simulink model "Hexapod_PD"  (R2026a)
settings: Solver=daessc  StopTime=ref.t(end)  FixedStep=2e-5
InitFcn:
  | startup
model workspace: external: MATLAB File Hexapod_DataFile.m (data not in the file)
undefined symbols (not defined in the file or in its folder): ref, robot, smiData, vc, X, Y, Z
libraries: sm_lib x805, nesl_utility x43
(part 11 of 15)

== system Hexapod_PD/Base/Base_Side_a_2_RIGID/x90576A137_Medium_Strength_Steel_Nylon_Insert_Locknut_2_RIGID ==
  ReferenceFrame : sm_lib/Frames and Transforms/Reference Frame
  Solid : sm_lib/Body Elements/File Solid  ExtGeomFileName=90576A137_Medium-Strength Steel Nylon-Insert Locknut_90576A137_sldprt.STEP  UnitType=FromFile  ExtGeomFileUnits=m  StepReaderType=HEX  ExportConvexHullGeometry=off  InertiaType=Custom  BasedOnType=DensityFromFile  Density=1000  DensityUnits=kg/m^3  Mass=smiData.Solid(5).mass  MassUnits=kg  CenterOfMass=smiData.Solid(5).CoM  CenterOfMassUnits=mm  MomentsOfInertia=smiData.Solid(5).MoI  MomentsOfInertiaUnits=kg*mm^2  ProductsOfInertia=smiData.Solid(5).PoI  ProductsOfInertiaUnits=kg*mm^2  GraphicType=FromGeometry  MarkerShape=Sphere  MarkerSize=10  GraphicVisPropType=SimpleVisualProperties  GraphicDiffuseColor=smiData.Solid(5).color  GraphicOpacity=smiData.Solid(5).opacity  GraphicSpecularColor=[0.5 0.5 0.5 1.0]  GraphicAmbientColor=[0.15 0.15 0.15 1.0]  GraphicEmissiveColor=[0.0 0.0 0.0 1.0]  GraphicShininess=75  DoExposeReferenceFrame=on  SerializedFrames=<Frames/>
  F : PMIOPort  Side=Left
  connections:
  Solid/RConn1 -- ReferenceFrame/RConn1 -- F/RConn1

== system Hexapod_PD/Base/Base_Side_a_2_RIGID/x90576A137_Medium_Strength_Steel_Nylon_Insert_Locknut_3_RIGID ==
  ReferenceFrame : sm_lib/Frames and Transforms/Reference Frame
  Solid : sm_lib/Body Elements/File Solid  ExtGeomFileName=90576A137_Medium-Strength Steel Nylon-Insert Locknut_90576A137_sldprt.STEP  UnitType=FromFile  ExtGeomFileUnits=m  StepReaderType=HEX  ExportConvexHullGeometry=off  InertiaType=Custom  BasedOnType=DensityFromFile  Density=1000  DensityUnits=kg/m^3  Mass=smiData.Solid(5).mass  MassUnits=kg  CenterOfMass=smiData.Solid(5).CoM  CenterOfMassUnits=mm  MomentsOfInertia=smiData.Solid(5).MoI  MomentsOfInertiaUnits=kg*mm^2  ProductsOfInertia=smiData.Solid(5).PoI  ProductsOfInertiaUnits=kg*mm^2  GraphicType=FromGeometry  MarkerShape=Sphere  MarkerSize=10  GraphicVisPropType=SimpleVisualProperties  GraphicDiffuseColor=smiData.Solid(5).color  GraphicOpacity=smiData.Solid(5).opacity  GraphicSpecularColor=[0.5 0.5 0.5 1.0]  GraphicAmbientColor=[0.15 0.15 0.15 1.0]  GraphicEmissiveColor=[0.0 0.0 0.0 1.0]  GraphicShininess=75  DoExposeReferenceFrame=on  SerializedFrames=<Frames/>
  F : PMIOPort  Side=Left
  connections:
  Solid/RConn1 -- ReferenceFrame/RConn1 -- F/RConn1

== system Hexapod_PD/Base/Base_Side_a_2_RIGID/x90576A137_Medium_Strength_Steel_Nylon_Insert_Locknut_4_RIGID ==
  ReferenceFrame : sm_lib/Frames and Transforms/Reference Frame
  Solid : sm_lib/Body Elements/File Solid  ExtGeomFileName=90576A137_Medium-Strength Steel Nylon-Insert Locknut_90576A137_sldprt.STEP  UnitType=FromFile  ExtGeomFileUnits=m  StepReaderType=HEX  ExportConvexHullGeometry=off  InertiaType=Custom  BasedOnType=DensityFromFile  Density=1000  DensityUnits=kg/m^3  Mass=smiData.Solid(5).mass  MassUnits=kg  CenterOfMass=smiData.Solid(5).CoM  CenterOfMassUnits=mm  MomentsOfInertia=smiData.Solid(5).MoI  MomentsOfInertiaUnits=kg*mm^2  ProductsOfInertia=smiData.Solid(5).PoI  ProductsOfInertiaUnits=kg*mm^2  GraphicType=FromGeometry  MarkerShape=Sphere  MarkerSize=10  GraphicVisPropType=SimpleVisualProperties  GraphicDiffuseColor=smiData.Solid(5).color  GraphicOpacity=smiData.Solid(5).opacity  GraphicSpecularColor=[0.5 0.5 0.5 1.0]  GraphicAmbientColor=[0.15 0.15 0.15 1.0]  GraphicEmissiveColor=[0.0 0.0 0.0 1.0]  GraphicShininess=75  DoExposeReferenceFrame=on  SerializedFrames=<Frames/>
  F : PMIOPort  Side=Left
  connections:
  Solid/RConn1 -- ReferenceFrame/RConn1 -- F/RConn1

== system Hexapod_PD/Base/Base_Side_a_2_RIGID/x91259A710_Alloy_Steel_Shoulder_Screw_1_RIGID ==
  ReferenceFrame : sm_lib/Frames and Transforms/Reference Frame
  Solid : sm_lib/Body Elements/File Solid  ExtGeomFileName=91259A710_Alloy Steel Shoulder Screw_91259A710_sldprt.STEP  UnitType=FromFile  ExtGeomFileUnits=m  StepReaderType=HEX  ExportConvexHullGeometry=off  InertiaType=Custom  BasedOnType=DensityFromFile  Density=1000  DensityUnits=kg/m^3  Mass=smiData.Solid(4).mass  MassUnits=kg  CenterOfMass=smiData.Solid(4).CoM  CenterOfMassUnits=in  MomentsOfInertia=smiData.Solid(4).MoI  MomentsOfInertiaUnits=kg*in^2  ProductsOfInertia=smiData.Solid(4).PoI  ProductsOfInertiaUnits=kg*in^2  GraphicType=FromGeometry  MarkerShape=Sphere  MarkerSize=10  GraphicVisPropType=SimpleVisualProperties  GraphicDiffuseColor=smiData.Solid(4).color  GraphicOpacity=smiData.Solid(4).opacity  GraphicSpecularColor=[0.5 0.5 0.5 1.0]  GraphicAmbientColor=[0.15 0.15 0.15 1.0]  GraphicEmissiveColor=[0.0 0.0 0.0 1.0]  GraphicShininess=75  DoExposeReferenceFrame=on  SerializedFrames=<Frames/>
  F : PMIOPort  Side=Left
  connections:
  Solid/RConn1 -- ReferenceFrame/RConn1 -- F/RConn1

== system Hexapod_PD/Base/Base_Side_a_2_RIGID/x91259A710_Alloy_Steel_Shoulder_Screw_2_RIGID ==
  ReferenceFrame : sm_lib/Frames and Transforms/Reference Frame
  Solid : sm_lib/Body Elements/File Solid  ExtGeomFileName=91259A710_Alloy Steel Shoulder Screw_91259A710_sldprt.STEP  UnitType=FromFile  ExtGeomFileUnits=m  StepReaderType=HEX  ExportConvexHullGeometry=off  InertiaType=Custom  BasedOnType=DensityFromFile  Density=1000  DensityUnits=kg/m^3  Mass=smiData.Solid(4).mass  MassUnits=kg  CenterOfMass=smiData.Solid(4).CoM  CenterOfMassUnits=in  MomentsOfInertia=smiData.Solid(4).MoI  MomentsOfInertiaUnits=kg*in^2  ProductsOfInertia=smiData.Solid(4).PoI  ProductsOfInertiaUnits=kg*in^2  GraphicType=FromGeometry  MarkerShape=Sphere  MarkerSize=10  GraphicVisPropType=SimpleVisualProperties  GraphicDiffuseColor=smiData.Solid(4).color  GraphicOpacity=smiData.Solid(4).opacity  GraphicSpecularColor=[0.5 0.5 0.5 1.0]  GraphicAmbientColor=[0.15 0.15 0.15 1.0]  GraphicEmissiveColor=[0.0 0.0 0.0 1.0]  GraphicShininess=75  DoExposeReferenceFrame=on  SerializedFrames=<Frames/>
  F : PMIOPort  Side=Left
  connections:
  Solid/RConn1 -- ReferenceFrame/RConn1 -- F/RConn1

== system Hexapod_PD/Base/Base_Side_a_2_RIGID/x91259A710_Alloy_Steel_Shoulder_Screw_3_RIGID ==
  ReferenceFrame : sm_lib/Frames and Transforms/Reference Frame
  Solid : sm_lib/Body Elements/File Solid  ExtGeomFileName=91259A710_Alloy Steel Shoulder Screw_91259A710_sldprt.STEP  UnitType=FromFile  ExtGeomFileUnits=m  StepReaderType=HEX  ExportConvexHullGeometry=off  InertiaType=Custom  BasedOnType=DensityFromFile  Density=1000  DensityUnits=kg/m^3  Mass=smiData.Solid(4).mass  MassUnits=kg  CenterOfMass=smiData.Solid(4).CoM  CenterOfMassUnits=in  MomentsOfInertia=smiData.Solid(4).MoI  MomentsOfInertiaUnits=kg*in^2  ProductsOfInertia=smiData.Solid(4).PoI  ProductsOfInertiaUnits=kg*in^2  GraphicType=FromGeometry  MarkerShape=Sphere  MarkerSize=10  GraphicVisPropType=SimpleVisualProperties  GraphicDiffuseColor=smiData.Solid(4).color  GraphicOpacity=smiData.Solid(4).opacity  GraphicSpecularColor=[0.5 0.5 0.5 1.0]  GraphicAmbientColor=[0.15 0.15 0.15 1.0]  GraphicEmissiveColor=[0.0 0.0 0.0 1.0]  GraphicShininess=75  DoExposeReferenceFrame=on  SerializedFrames=<Frames/>
  F : PMIOPort  Side=Left
  connections:
  Solid/RConn1 -- ReferenceFrame/RConn1 -- F/RConn1

== system Hexapod_PD/Base/Base_Side_a_2_RIGID/x91259A710_Alloy_Steel_Shoulder_Screw_4_RIGID ==
  ReferenceFrame : sm_lib/Frames and Transforms/Reference Frame
  Solid : sm_lib/Body Elements/File Solid  ExtGeomFileName=91259A710_Alloy Steel Shoulder Screw_91259A710_sldprt.STEP  UnitType=FromFile  ExtGeomFileUnits=m  StepReaderType=HEX  ExportConvexHullGeometry=off  InertiaType=Custom  BasedOnType=DensityFromFile  Density=1000  DensityUnits=kg/m^3  Mass=smiData.Solid(4).mass  MassUnits=kg  CenterOfMass=smiData.Solid(4).CoM  CenterOfMassUnits=in  MomentsOfInertia=smiData.Solid(4).MoI  MomentsOfInertiaUnits=kg*in^2  ProductsOfInertia=smiData.Solid(4).PoI  ProductsOfInertiaUnits=kg*in^2  GraphicType=FromGeometry  MarkerShape=Sphere  MarkerSize=10  GraphicVisPropType=SimpleVisualProperties  GraphicDiffuseColor=smiData.Solid(4).color  GraphicOpacity=smiData.Solid(4).opacity  GraphicSpecularColor=[0.5 0.5 0.5 1.0]  GraphicAmbientColor=[0.15 0.15 0.15 1.0]  GraphicEmissiveColor=[0.0 0.0 0.0 1.0]  GraphicShininess=75  DoExposeReferenceFrame=on  SerializedFrames=<Frames/>
  F : PMIOPort  Side=Left
  connections:
  Solid/RConn1 -- ReferenceFrame/RConn1 -- F/RConn1

== system Hexapod_PD/Base/Base_Side_a_2_RIGID/x91259A710_Alloy_Steel_Shoulder_Screw_5_RIGID ==
  ReferenceFrame : sm_lib/Frames and Transforms/Reference Frame
  Solid : sm_lib/Body Elements/File Solid  ExtGeomFileName=91259A710_Alloy Steel Shoulder Screw_91259A710_sldprt.STEP  UnitType=FromFile  ExtGeomFileUnits=m  StepReaderType=HEX  ExportConvexHullGeometry=off  InertiaType=Custom  BasedOnType=DensityFromFile  Density=1000  DensityUnits=kg/m^3  Mass=smiData.Solid(4).mass  MassUnits=kg  CenterOfMass=smiData.Solid(4).CoM  CenterOfMassUnits=in  MomentsOfInertia=smiData.Solid(4).MoI  MomentsOfInertiaUnits=kg*in^2  ProductsOfInertia=smiData.Solid(4).PoI  ProductsOfInertiaUnits=kg*in^2  GraphicType=FromGeometry  MarkerShape=Sphere  MarkerSize=10  GraphicVisPropType=SimpleVisualProperties  GraphicDiffuseColor=smiData.Solid(4).color  GraphicOpacity=smiData.Solid(4).opacity  GraphicSpecularColor=[0.5 0.5 0.5 1.0]  GraphicAmbientColor=[0.15 0.15 0.15 1.0]  GraphicEmissiveColor=[0.0 0.0 0.0 1.0]  GraphicShininess=75  DoExposeReferenceFrame=on  SerializedFrames=<Frames/>
  F : PMIOPort  Side=Left
  connections:
  Solid/RConn1 -- ReferenceFrame/RConn1 -- F/RConn1

== system Hexapod_PD/Base/Base_Side_a_2_RIGID/x91259A710_Alloy_Steel_Shoulder_Screw_6_RIGID ==
  ReferenceFrame : sm_lib/Frames and Transforms/Reference Frame
  Solid : sm_lib/Body Elements/File Solid  ExtGeomFileName=91259A710_Alloy Steel Shoulder Screw_91259A710_sldprt.STEP  UnitType=FromFile  ExtGeomFileUnits=m  StepReaderType=HEX  ExportConvexHullGeometry=off  InertiaType=Custom  BasedOnType=DensityFromFile  Density=1000  DensityUnits=kg/m^3  Mass=smiData.Solid(4).mass  MassUnits=kg  CenterOfMass=smiData.Solid(4).CoM  CenterOfMassUnits=in  MomentsOfInertia=smiData.Solid(4).MoI  MomentsOfInertiaUnits=kg*in^2  ProductsOfInertia=smiData.Solid(4).PoI  ProductsOfInertiaUnits=kg*in^2  GraphicType=FromGeometry  MarkerShape=Sphere  MarkerSize=10  GraphicVisPropType=SimpleVisualProperties  GraphicDiffuseColor=smiData.Solid(4).color  GraphicOpacity=smiData.Solid(4).opacity  GraphicSpecularColor=[0.5 0.5 0.5 1.0]  GraphicAmbientColor=[0.15 0.15 0.15 1.0]  GraphicEmissiveColor=[0.0 0.0 0.0 1.0]  GraphicShininess=75  DoExposeReferenceFrame=on  SerializedFrames=<Frames/>
  F : PMIOPort  Side=Left
  connections:
  Solid/RConn1 -- ReferenceFrame/RConn1 -- F/RConn1

== system Hexapod_PD/Base/Base_Side_a_2_RIGID/x91259A710_Alloy_Steel_Shoulder_Screw_7_RIGID ==
  ReferenceFrame : sm_lib/Frames and Transforms/Reference Frame
  Solid : sm_lib/Body Elements/File Solid  ExtGeomFileName=91259A710_Alloy Steel Shoulder Screw_91259A710_sldprt.STEP  UnitType=FromFile  ExtGeomFileUnits=m  StepReaderType=HEX  ExportConvexHullGeometry=off  InertiaType=Custom  BasedOnType=DensityFromFile  Density=1000  DensityUnits=kg/m^3  Mass=smiData.Solid(4).mass  MassUnits=kg  CenterOfMass=smiData.Solid(4).CoM  CenterOfMassUnits=in  MomentsOfInertia=smiData.Solid(4).MoI  MomentsOfInertiaUnits=kg*in^2  ProductsOfInertia=smiData.Solid(4).PoI  ProductsOfInertiaUnits=kg*in^2  GraphicType=FromGeometry  MarkerShape=Sphere  MarkerSize=10  GraphicVisPropType=SimpleVisualProperties  GraphicDiffuseColor=smiData.Solid(4).color  GraphicOpacity=smiData.Solid(4).opacity  GraphicSpecularColor=[0.5 0.5 0.5 1.0]  GraphicAmbientColor=[0.15 0.15 0.15 1.0]  GraphicEmissiveColor=[0.0 0.0 0.0 1.0]  GraphicShininess=75  DoExposeReferenceFrame=on  SerializedFrames=<Frames/>
  F : PMIOPort  Side=Left
  connections:
  Solid/RConn1 -- ReferenceFrame/RConn1 -- F/RConn1

== system Hexapod_PD/Base/Base_Side_a_2_RIGID/x91259A710_Alloy_Steel_Shoulder_Screw_8_RIGID ==
  ReferenceFrame : sm_lib/Frames and Transforms/Reference Frame
  Solid : sm_lib/Body Elements/File Solid  ExtGeomFileName=91259A710_Alloy Steel Shoulder Screw_91259A710_sldprt.STEP  UnitType=FromFile  ExtGeomFileUnits=m  StepReaderType=HEX  ExportConvexHullGeometry=off  InertiaType=Custom  BasedOnType=DensityFromFile  Density=1000  DensityUnits=kg/m^3  Mass=smiData.Solid(4).mass  MassUnits=kg  CenterOfMass=smiData.Solid(4).CoM  CenterOfMassUnits=in  MomentsOfInertia=smiData.Solid(4).MoI  MomentsOfInertiaUnits=kg*in^2  ProductsOfInertia=smiData.Solid(4).PoI  ProductsOfInertiaUnits=kg*in^2  GraphicType=FromGeometry  MarkerShape=Sphere  MarkerSize=10  GraphicVisPropType=SimpleVisualProperties  GraphicDiffuseColor=smiData.Solid(4).color  GraphicOpacity=smiData.Solid(4).opacity  GraphicSpecularColor=[0.5 0.5 0.5 1.0]  GraphicAmbientColor=[0.15 0.15 0.15 1.0]  GraphicEmissiveColor=[0.0 0.0 0.0 1.0]  GraphicShininess=75  DoExposeReferenceFrame=on  SerializedFrames=<Frames/>
  F : PMIOPort  Side=Left
  connections:
  Solid/RConn1 -- ReferenceFrame/RConn1 -- F/RConn1

== system Hexapod_PD/Base/Base_Side_a_2_RIGID/x91273A784_Same_Size_Thread_18_8_Stainless_Steel_Shoulder_Screw_10_RIGID ==
  ReferenceFrame : sm_lib/Frames and Transforms/Reference Frame
  Solid : sm_lib/Body Elements/File Solid  ExtGeomFileName=91273A784_Same-Size Thread 18-8 Stainless Steel Shoulder Screw_91273A784_sldprt.STEP  UnitType=FromFile  ExtGeomFileUnits=m  StepReaderType=HEX  ExportConvexHullGeometry=off  InertiaType=Custom  BasedOnType=DensityFromFile  Density=1000  DensityUnits=kg/m^3  Mass=smiData.Solid(10).mass  MassUnits=kg  CenterOfMass=smiData.Solid(10).CoM  CenterOfMassUnits=mm  MomentsOfInertia=smiData.Solid(10).MoI  MomentsOfInertiaUnits=kg*mm^2  ProductsOfInertia=smiData.Solid(10).PoI  ProductsOfInertiaUnits=kg*mm^2  GraphicType=FromGeometry  MarkerShape=Sphere  MarkerSize=10  GraphicVisPropType=SimpleVisualProperties  GraphicDiffuseColor=smiData.Solid(10).color  GraphicOpacity=smiData.Solid(10).opacity  GraphicSpecularColor=[0.5 0.5 0.5 1.0]  GraphicAmbientColor=[0.15 0.15 0.15 1.0]  GraphicEmissiveColor=[0.0 0.0 0.0 1.0]  GraphicShininess=75  DoExposeReferenceFrame=on  SerializedFrames=<Frames/>
  F : PMIOPort  Side=Left
  connections:
  Solid/RConn1 -- ReferenceFrame/RConn1 -- F/RConn1

== system Hexapod_PD/Base/Base_Side_a_2_RIGID/x91273A784_Same_Size_Thread_18_8_Stainless_Steel_Shoulder_Screw_11_RIGID ==
  ReferenceFrame : sm_lib/Frames and Transforms/Reference Frame
  Solid : sm_lib/Body Elements/File Solid  ExtGeomFileName=91273A784_Same-Size Thread 18-8 Stainless Steel Shoulder Screw_91273A784_sldprt.STEP  UnitType=FromFile  ExtGeomFileUnits=m  StepReaderType=HEX  ExportConvexHullGeometry=off  InertiaType=Custom  BasedOnType=DensityFromFile  Density=1000  DensityUnits=kg/m^3  Mass=smiData.Solid(10).mass  MassUnits=kg  CenterOfMass=smiData.Solid(10).CoM  CenterOfMassUnits=mm  MomentsOfInertia=smiData.Solid(10).MoI  MomentsOfInertiaUnits=kg*mm^2  ProductsOfInertia=smiData.Solid(10).PoI  ProductsOfInertiaUnits=kg*mm^2  GraphicType=FromGeometry  MarkerShape=Sphere  MarkerSize=10  GraphicVisPropType=SimpleVisualProperties  GraphicDiffuseColor=smiData.Solid(10).color  GraphicOpacity=smiData.Solid(10).opacity  GraphicSpecularColor=[0.5 0.5 0.5 1.0]  GraphicAmbientColor=[0.15 0.15 0.15 1.0]  GraphicEmissiveColor=[0.0 0.0 0.0 1.0]  GraphicShininess=75  DoExposeReferenceFrame=on  SerializedFrames=<Frames/>
  F : PMIOPort  Side=Left
  connections:
  Solid/RConn1 -- ReferenceFrame/RConn1 -- F/RConn1

== system Hexapod_PD/Base/Base_Side_a_2_RIGID/x91273A784_Same_Size_Thread_18_8_Stainless_Steel_Shoulder_Screw_12_RIGID ==
  ReferenceFrame : sm_lib/Frames and Transforms/Reference Frame
  Solid : sm_lib/Body Elements/File Solid  ExtGeomFileName=91273A784_Same-Size Thread 18-8 Stainless Steel Shoulder Screw_91273A784_sldprt.STEP  UnitType=FromFile  ExtGeomFileUnits=m  StepReaderType=HEX  ExportConvexHullGeometry=off  InertiaType=Custom  BasedOnType=DensityFromFile  Density=1000  DensityUnits=kg/m^3  Mass=smiData.Solid(10).mass  MassUnits=kg  CenterOfMass=smiData.Solid(10).CoM  CenterOfMassUnits=mm  MomentsOfInertia=smiData.Solid(10).MoI  MomentsOfInertiaUnits=kg*mm^2  ProductsOfInertia=smiData.Solid(10).PoI  ProductsOfInertiaUnits=kg*mm^2  GraphicType=FromGeometry  MarkerShape=Sphere  MarkerSize=10  GraphicVisPropType=SimpleVisualProperties  GraphicDiffuseColor=smiData.Solid(10).color  GraphicOpacity=smiData.Solid(10).opacity  GraphicSpecularColor=[0.5 0.5 0.5 1.0]  GraphicAmbientColor=[0.15 0.15 0.15 1.0]  GraphicEmissiveColor=[0.0 0.0 0.0 1.0]  GraphicShininess=75  DoExposeReferenceFrame=on  SerializedFrames=<Frames/>
  F : PMIOPort  Side=Left
  connections:
  Solid/RConn1 -- ReferenceFrame/RConn1 -- F/RConn1

== system Hexapod_PD/Base/Base_Side_a_2_RIGID/x91273A784_Same_Size_Thread_18_8_Stainless_Steel_Shoulder_Screw_13_RIGID ==
  ReferenceFrame : sm_lib/Frames and Transforms/Reference Frame
  Solid : sm_lib/Body Elements/File Solid  ExtGeomFileName=91273A784_Same-Size Thread 18-8 Stainless Steel Shoulder Screw_91273A784_sldprt.STEP  UnitType=FromFile  ExtGeomFileUnits=m  StepReaderType=HEX  ExportConvexHullGeometry=off  InertiaType=Custom  BasedOnType=DensityFromFile  Density=1000  DensityUnits=kg/m^3  Mass=smiData.Solid(10).mass  MassUnits=kg  CenterOfMass=smiData.Solid(10).CoM  CenterOfMassUnits=mm  MomentsOfInertia=smiData.Solid(10).MoI  MomentsOfInertiaUnits=kg*mm^2  ProductsOfInertia=smiData.Solid(10).PoI  ProductsOfInertiaUnits=kg*mm^2  GraphicType=FromGeometry  MarkerShape=Sphere  MarkerSize=10  GraphicVisPropType=SimpleVisualProperties  GraphicDiffuseColor=smiData.Solid(10).color  GraphicOpacity=smiData.Solid(10).opacity  GraphicSpecularColor=[0.5 0.5 0.5 1.0]  GraphicAmbientColor=[0.15 0.15 0.15 1.0]  GraphicEmissiveColor=[0.0 0.0 0.0 1.0]  GraphicShininess=75  DoExposeReferenceFrame=on  SerializedFrames=<Frames/>
  F : PMIOPort  Side=Left
  connections:
  Solid/RConn1 -- ReferenceFrame/RConn1 -- F/RConn1

== system Hexapod_PD/Base/Base_Side_a_2_RIGID/x91273A784_Same_Size_Thread_18_8_Stainless_Steel_Shoulder_Screw_14_RIGID ==
  ReferenceFrame : sm_lib/Frames and Transforms/Reference Frame
  Solid : sm_lib/Body Elements/File Solid  ExtGeomFileName=91273A784_Same-Size Thread 18-8 Stainless Steel Shoulder Screw_91273A784_sldprt.STEP  UnitType=FromFile  ExtGeomFileUnits=m  StepReaderType=HEX  ExportConvexHullGeometry=off  InertiaType=Custom  BasedOnType=DensityFromFile  Density=1000  DensityUnits=kg/m^3  Mass=smiData.Solid(10).mass  MassUnits=kg  CenterOfMass=smiData.Solid(10).CoM  CenterOfMassUnits=mm  MomentsOfInertia=smiData.Solid(10).MoI  MomentsOfInertiaUnits=kg*mm^2  ProductsOfInertia=smiData.Solid(10).PoI  ProductsOfInertiaUnits=kg*mm^2  GraphicType=FromGeometry  MarkerShape=Sphere  MarkerSize=10  GraphicVisPropType=SimpleVisualProperties  GraphicDiffuseColor=smiData.Solid(10).color  GraphicOpacity=smiData.Solid(10).opacity  GraphicSpecularColor=[0.5 0.5 0.5 1.0]  GraphicAmbientColor=[0.15 0.15 0.15 1.0]  GraphicEmissiveColor=[0.0 0.0 0.0 1.0]  GraphicShininess=75  DoExposeReferenceFrame=on  SerializedFrames=<Frames/>
  F : PMIOPort  Side=Left
  connections:
  Solid/RConn1 -- ReferenceFrame/RConn1 -- F/RConn1

== system Hexapod_PD/Base/Base_Side_a_2_RIGID/x91273A784_Same_Size_Thread_18_8_Stainless_Steel_Shoulder_Screw_1_RIGID ==
  ReferenceFrame : sm_lib/Frames and Transforms/Reference Frame
  Solid : sm_lib/Body Elements/File Solid  ExtGeomFileName=91273A784_Same-Size Thread 18-8 Stainless Steel Shoulder Screw_91273A784_sldprt.STEP  UnitType=FromFile  ExtGeomFileUnits=m  StepReaderType=HEX  ExportConvexHullGeometry=off  InertiaType=Custom  BasedOnType=DensityFromFile  Density=1000  DensityUnits=kg/m^3  Mass=smiData.Solid(10).mass  MassUnits=kg  CenterOfMass=smiData.Solid(10).CoM  CenterOfMassUnits=mm  MomentsOfInertia=smiData.Solid(10).MoI  MomentsOfInertiaUnits=kg*mm^2  ProductsOfInertia=smiData.Solid(10).PoI  ProductsOfInertiaUnits=kg*mm^2  GraphicType=FromGeometry  MarkerShape=Sphere  MarkerSize=10  GraphicVisPropType=SimpleVisualProperties  GraphicDiffuseColor=smiData.Solid(10).color  GraphicOpacity=smiData.Solid(10).opacity  GraphicSpecularColor=[0.5 0.5 0.5 1.0]  GraphicAmbientColor=[0.15 0.15 0.15 1.0]  GraphicEmissiveColor=[0.0 0.0 0.0 1.0]  GraphicShininess=75  DoExposeReferenceFrame=on  SerializedFrames=<Frames/>
  F : PMIOPort  Side=Left
  connections:
  Solid/RConn1 -- ReferenceFrame/RConn1 -- F/RConn1

== system Hexapod_PD/Base/Base_Side_a_2_RIGID/x91273A784_Same_Size_Thread_18_8_Stainless_Steel_Shoulder_Screw_2_RIGID ==
  ReferenceFrame : sm_lib/Frames and Transforms/Reference Frame
  Solid : sm_lib/Body Elements/File Solid  ExtGeomFileName=91273A784_Same-Size Thread 18-8 Stainless Steel Shoulder Screw_91273A784_sldprt.STEP  UnitType=FromFile  ExtGeomFileUnits=m  StepReaderType=HEX  ExportConvexHullGeometry=off  InertiaType=Custom  BasedOnType=DensityFromFile  Density=1000  DensityUnits=kg/m^3  Mass=smiData.Solid(10).mass  MassUnits=kg  CenterOfMass=smiData.Solid(10).CoM  CenterOfMassUnits=mm  MomentsOfInertia=smiData.Solid(10).MoI  MomentsOfInertiaUnits=kg*mm^2  ProductsOfInertia=smiData.Solid(10).PoI  ProductsOfInertiaUnits=kg*mm^2  GraphicType=FromGeometry  MarkerShape=Sphere  MarkerSize=10  GraphicVisPropType=SimpleVisualProperties  GraphicDiffuseColor=smiData.Solid(10).color  GraphicOpacity=smiData.Solid(10).opacity  GraphicSpecularColor=[0.5 0.5 0.5 1.0]  GraphicAmbientColor=[0.15 0.15 0.15 1.0]  GraphicEmissiveColor=[0.0 0.0 0.0 1.0]  GraphicShininess=75  DoExposeReferenceFrame=on  SerializedFrames=<Frames/>
  F : PMIOPort  Side=Left
  connections:
  Solid/RConn1 -- ReferenceFrame/RConn1 -- F/RConn1

== system Hexapod_PD/Base/Base_Side_a_2_RIGID/x91273A784_Same_Size_Thread_18_8_Stainless_Steel_Shoulder_Screw_3_RIGID ==
  ReferenceFrame : sm_lib/Frames and Transforms/Reference Frame
  Solid : sm_lib/Body Elements/File Solid  ExtGeomFileName=91273A784_Same-Size Thread 18-8 Stainless Steel Shoulder Screw_91273A784_sldprt.STEP  UnitType=FromFile  ExtGeomFileUnits=m  StepReaderType=HEX  ExportConvexHullGeometry=off  InertiaType=Custom  BasedOnType=DensityFromFile  Density=1000  DensityUnits=kg/m^3  Mass=smiData.Solid(10).mass  MassUnits=kg  CenterOfMass=smiData.Solid(10).CoM  CenterOfMassUnits=mm  MomentsOfInertia=smiData.Solid(10).MoI  MomentsOfInertiaUnits=kg*mm^2  ProductsOfInertia=smiData.Solid(10).PoI  ProductsOfInertiaUnits=kg*mm^2  GraphicType=FromGeometry  MarkerShape=Sphere  MarkerSize=10  GraphicVisPropType=SimpleVisualProperties  GraphicDiffuseColor=smiData.Solid(10).color  GraphicOpacity=smiData.Solid(10).opacity  GraphicSpecularColor=[0.5 0.5 0.5 1.0]  GraphicAmbientColor=[0.15 0.15 0.15 1.0]  GraphicEmissiveColor=[0.0 0.0 0.0 1.0]  GraphicShininess=75  DoExposeReferenceFrame=on  SerializedFrames=<Frames/>
  F : PMIOPort  Side=Left
  connections:
  Solid/RConn1 -- ReferenceFrame/RConn1 -- F/RConn1

== system Hexapod_PD/Base/Base_Side_a_2_RIGID/x91273A784_Same_Size_Thread_18_8_Stainless_Steel_Shoulder_Screw_4_RIGID ==
  ReferenceFrame : sm_lib/Frames and Transforms/Reference Frame
  Solid : sm_lib/Body Elements/File Solid  ExtGeomFileName=91273A784_Same-Size Thread 18-8 Stainless Steel Shoulder Screw_91273A784_sldprt.STEP  UnitType=FromFile  ExtGeomFileUnits=m  StepReaderType=HEX  ExportConvexHullGeometry=off  InertiaType=Custom  BasedOnType=DensityFromFile  Density=1000  DensityUnits=kg/m^3  Mass=smiData.Solid(10).mass  MassUnits=kg  CenterOfMass=smiData.Solid(10).CoM  CenterOfMassUnits=mm  MomentsOfInertia=smiData.Solid(10).MoI  MomentsOfInertiaUnits=kg*mm^2  ProductsOfInertia=smiData.Solid(10).PoI  ProductsOfInertiaUnits=kg*mm^2  GraphicType=FromGeometry  MarkerShape=Sphere  MarkerSize=10  GraphicVisPropType=SimpleVisualProperties  GraphicDiffuseColor=smiData.Solid(10).color  GraphicOpacity=smiData.Solid(10).opacity  GraphicSpecularColor=[0.5 0.5 0.5 1.0]  GraphicAmbientColor=[0.15 0.15 0.15 1.0]  GraphicEmissiveColor=[0.0 0.0 0.0 1.0]  GraphicShininess=75  DoExposeReferenceFrame=on  SerializedFrames=<Frames/>
  F : PMIOPort  Side=Left
  connections:
  Solid/RConn1 -- ReferenceFrame/RConn1 -- F/RConn1

== system Hexapod_PD/Base/Base_Side_a_2_RIGID/x91273A784_Same_Size_Thread_18_8_Stainless_Steel_Shoulder_Screw_5_RIGID ==
  ReferenceFrame : sm_lib/Frames and Transforms/Reference Frame
  Solid : sm_lib/Body Elements/File Solid  ExtGeomFileName=91273A784_Same-Size Thread 18-8 Stainless Steel Shoulder Screw_91273A784_sldprt.STEP  UnitType=FromFile  ExtGeomFileUnits=m  StepReaderType=HEX  ExportConvexHullGeometry=off  InertiaType=Custom  BasedOnType=DensityFromFile  Density=1000  DensityUnits=kg/m^3  Mass=smiData.Solid(10).mass  MassUnits=kg  CenterOfMass=smiData.Solid(10).CoM  CenterOfMassUnits=mm  MomentsOfInertia=smiData.Solid(10).MoI  MomentsOfInertiaUnits=kg*mm^2  ProductsOfInertia=smiData.Solid(10).PoI  ProductsOfInertiaUnits=kg*mm^2  GraphicType=FromGeometry  MarkerShape=Sphere  MarkerSize=10  GraphicVisPropType=SimpleVisualProperties  GraphicDiffuseColor=smiData.Solid(10).color  GraphicOpacity=smiData.Solid(10).opacity  GraphicSpecularColor=[0.5 0.5 0.5 1.0]  GraphicAmbientColor=[0.15 0.15 0.15 1.0]  GraphicEmissiveColor=[0.0 0.0 0.0 1.0]  GraphicShininess=75  DoExposeReferenceFrame=on  SerializedFrames=<Frames/>
  F : PMIOPort  Side=Left
  connections:
  Solid/RConn1 -- ReferenceFrame/RConn1 -- F/RConn1

== system Hexapod_PD/Base/Base_Side_a_2_RIGID/x91273A784_Same_Size_Thread_18_8_Stainless_Steel_Shoulder_Screw_6_RIGID ==
  ReferenceFrame : sm_lib/Frames and Transforms/Reference Frame
  Solid : sm_lib/Body Elements/File Solid  ExtGeomFileName=91273A784_Same-Size Thread 18-8 Stainless Steel Shoulder Screw_91273A784_sldprt.STEP  UnitType=FromFile  ExtGeomFileUnits=m  StepReaderType=HEX  ExportConvexHullGeometry=off  InertiaType=Custom  BasedOnType=DensityFromFile  Density=1000  DensityUnits=kg/m^3  Mass=smiData.Solid(10).mass  MassUnits=kg  CenterOfMass=smiData.Solid(10).CoM  CenterOfMassUnits=mm  MomentsOfInertia=smiData.Solid(10).MoI  MomentsOfInertiaUnits=kg*mm^2  ProductsOfInertia=smiData.Solid(10).PoI  ProductsOfInertiaUnits=kg*mm^2  GraphicType=FromGeometry  MarkerShape=Sphere  MarkerSize=10  GraphicVisPropType=SimpleVisualProperties  GraphicDiffuseColor=smiData.Solid(10).color  GraphicOpacity=smiData.Solid(10).opacity  GraphicSpecularColor=[0.5 0.5 0.5 1.0]  GraphicAmbientColor=[0.15 0.15 0.15 1.0]  GraphicEmissiveColor=[0.0 0.0 0.0 1.0]  GraphicShininess=75  DoExposeReferenceFrame=on  SerializedFrames=<Frames/>
  F : PMIOPort  Side=Left
  connections:
  Solid/RConn1 -- ReferenceFrame/RConn1 -- F/RConn1

== system Hexapod_PD/Base/Base_Side_a_2_RIGID/x91273A784_Same_Size_Thread_18_8_Stainless_Steel_Shoulder_Screw_7_RIGID ==
  ReferenceFrame : sm_lib/Frames and Transforms/Reference Frame
  Solid : sm_lib/Body Elements/File Solid  ExtGeomFileName=91273A784_Same-Size Thread 18-8 Stainless Steel Shoulder Screw_91273A784_sldprt.STEP  UnitType=FromFile  ExtGeomFileUnits=m  StepReaderType=HEX  ExportConvexHullGeometry=off  InertiaType=Custom  BasedOnType=DensityFromFile  Density=1000  DensityUnits=kg/m^3  Mass=smiData.Solid(10).mass  MassUnits=kg  CenterOfMass=smiData.Solid(10).CoM  CenterOfMassUnits=mm  MomentsOfInertia=smiData.Solid(10).MoI  MomentsOfInertiaUnits=kg*mm^2  ProductsOfInertia=smiData.Solid(10).PoI  ProductsOfInertiaUnits=kg*mm^2  GraphicType=FromGeometry  MarkerShape=Sphere  MarkerSize=10  GraphicVisPropType=SimpleVisualProperties  GraphicDiffuseColor=smiData.Solid(10).color  GraphicOpacity=smiData.Solid(10).opacity  GraphicSpecularColor=[0.5 0.5 0.5 1.0]  GraphicAmbientColor=[0.15 0.15 0.15 1.0]  GraphicEmissiveColor=[0.0 0.0 0.0 1.0]  GraphicShininess=75  DoExposeReferenceFrame=on  SerializedFrames=<Frames/>
  F : PMIOPort  Side=Left
  connections:
  Solid/RConn1 -- ReferenceFrame/RConn1 -- F/RConn1

== system Hexapod_PD/Base/Base_Side_a_2_RIGID/x91273A784_Same_Size_Thread_18_8_Stainless_Steel_Shoulder_Screw_8_RIGID ==
  ReferenceFrame : sm_lib/Frames and Transforms/Reference Frame
  Solid : sm_lib/Body Elements/File Solid  ExtGeomFileName=91273A784_Same-Size Thread 18-8 Stainless Steel Shoulder Screw_91273A784_sldprt.STEP  UnitType=FromFile  ExtGeomFileUnits=m  StepReaderType=HEX  ExportConvexHullGeometry=off  InertiaType=Custom  BasedOnType=DensityFromFile  Density=1000  DensityUnits=kg/m^3  Mass=smiData.Solid(10).mass  MassUnits=kg  CenterOfMass=smiData.Solid(10).CoM  CenterOfMassUnits=mm  MomentsOfInertia=smiData.Solid(10).MoI  MomentsOfInertiaUnits=kg*mm^2  ProductsOfInertia=smiData.Solid(10).PoI  ProductsOfInertiaUnits=kg*mm^2  GraphicType=FromGeometry  MarkerShape=Sphere  MarkerSize=10  GraphicVisPropType=SimpleVisualProperties  GraphicDiffuseColor=smiData.Solid(10).color  GraphicOpacity=smiData.Solid(10).opacity  GraphicSpecularColor=[0.5 0.5 0.5 1.0]  GraphicAmbientColor=[0.15 0.15 0.15 1.0]  GraphicEmissiveColor=[0.0 0.0 0.0 1.0]  GraphicShininess=75  DoExposeReferenceFrame=on  SerializedFrames=<Frames/>
  F : PMIOPort  Side=Left
  connections:
  Solid/RConn1 -- ReferenceFrame/RConn1 -- F/RConn1

== system Hexapod_PD/Base/Base_Side_a_2_RIGID/x91273A784_Same_Size_Thread_18_8_Stainless_Steel_Shoulder_Screw_9_RIGID ==
  ReferenceFrame : sm_lib/Frames and Transforms/Reference Frame
  Solid : sm_lib/Body Elements/File Solid  ExtGeomFileName=91273A784_Same-Size Thread 18-8 Stainless Steel Shoulder Screw_91273A784_sldprt.STEP  UnitType=FromFile  ExtGeomFileUnits=m  StepReaderType=HEX  ExportConvexHullGeometry=off  InertiaType=Custom  BasedOnType=DensityFromFile  Density=1000  DensityUnits=kg/m^3  Mass=smiData.Solid(10).mass  MassUnits=kg  CenterOfMass=smiData.Solid(10).CoM  CenterOfMassUnits=mm  MomentsOfInertia=smiData.Solid(10).MoI  MomentsOfInertiaUnits=kg*mm^2  ProductsOfInertia=smiData.Solid(10).PoI  ProductsOfInertiaUnits=kg*mm^2  GraphicType=FromGeometry  MarkerShape=Sphere  MarkerSize=10  GraphicVisPropType=SimpleVisualProperties  GraphicDiffuseColor=smiData.Solid(10).color  GraphicOpacity=smiData.Solid(10).opacity  GraphicSpecularColor=[0.5 0.5 0.5 1.0]  GraphicAmbientColor=[0.15 0.15 0.15 1.0]  GraphicEmissiveColor=[0.0 0.0 0.0 1.0]  GraphicShininess=75  DoExposeReferenceFrame=on  SerializedFrames=<Frames/>
  F : PMIOPort  Side=Left
  connections:
  Solid/RConn1 -- ReferenceFrame/RConn1 -- F/RConn1

== system Hexapod_PD/Base/Base_Side_a_2_RIGID/x95245A233_Grade_B7_Medium_Strength_Steel_Threaded_Rod_1_RIGID ==
  ReferenceFrame : sm_lib/Frames and Transforms/Reference Frame
  Solid : sm_lib/Body Elements/File Solid  ExtGeomFileName=95245A233_Grade B7 Medium-Strength Steel Threaded Rod_95245A233_sldprt.STEP  UnitType=FromFile  ExtGeomFileUnits=m  StepReaderType=HEX  ExportConvexHullGeometry=off  InertiaType=Custom  BasedOnType=DensityFromFile  Density=1000  DensityUnits=kg/m^3  Mass=smiData.Solid(6).mass  MassUnits=kg  CenterOfMass=smiData.Solid(6).CoM  CenterOfMassUnits=mm  MomentsOfInertia=smiData.Solid(6).MoI  MomentsOfInertiaUnits=kg*mm^2  ProductsOfInertia=smiData.Solid(6).PoI  ProductsOfInertiaUnits=kg*mm^2  GraphicType=FromGeometry  MarkerShape=Sphere  MarkerSize=10  GraphicVisPropType=SimpleVisualProperties  GraphicDiffuseColor=smiData.Solid(6).color  GraphicOpacity=smiData.Solid(6).opacity  GraphicSpecularColor=[0.5 0.5 0.5 1.0]  GraphicAmbientColor=[0.15 0.15 0.15 1.0]  GraphicEmissiveColor=[0.0 0.0 0.0 1.0]  GraphicShininess=75  DoExposeReferenceFrame=on  SerializedFrames=<Frames/>
  F : PMIOPort  Side=Left
  connections:
  Solid/RConn1 -- ReferenceFrame/RConn1 -- F/RConn1

== system Hexapod_PD/Base/Base_Side_a_2_RIGID/x95245A233_Grade_B7_Medium_Strength_Steel_Threaded_Rod_2_RIGID ==
  ReferenceFrame : sm_lib/Frames and Transforms/Reference Frame
  Solid : sm_lib/Body Elements/File Solid  ExtGeomFileName=95245A233_Grade B7 Medium-Strength Steel Threaded Rod_95245A233_sldprt.STEP  UnitType=FromFile  ExtGeomFileUnits=m  StepReaderType=HEX  ExportConvexHullGeometry=off  InertiaType=Custom  BasedOnType=DensityFromFile  Density=1000  DensityUnits=kg/m^3  Mass=smiData.Solid(6).mass  MassUnits=kg  CenterOfMass=smiData.Solid(6).CoM  CenterOfMassUnits=mm  MomentsOfInertia=smiData.Solid(6).MoI  MomentsOfInertiaUnits=kg*mm^2  ProductsOfInertia=smiData.Solid(6).PoI  ProductsOfInertiaUnits=kg*mm^2  GraphicType=FromGeometry  MarkerShape=Sphere  MarkerSize=10  GraphicVisPropType=SimpleVisualProperties  GraphicDiffuseColor=smiData.Solid(6).color  GraphicOpacity=smiData.Solid(6).opacity  GraphicSpecularColor=[0.5 0.5 0.5 1.0]  GraphicAmbientColor=[0.15 0.15 0.15 1.0]  GraphicEmissiveColor=[0.0 0.0 0.0 1.0]  GraphicShininess=75  DoExposeReferenceFrame=on  SerializedFrames=<Frames/>
  F : PMIOPort  Side=Left
  connections:
  Solid/RConn1 -- ReferenceFrame/RConn1 -- F/RConn1

== system Hexapod_PD/Base/Base_Side_a_3_RIGID/MotorStator_1_RIGID ==
  ReferenceFrame : sm_lib/Frames and Transforms/Reference Frame
  Solid : sm_lib/Body Elements/File Solid  ExtGeomFileName=MotorStator_Default_sldprt.STEP  UnitType=FromFile  ExtGeomFileUnits=m  StepReaderType=HEX  ExportConvexHullGeometry=off  InertiaType=Custom  BasedOnType=DensityFromFile  Density=1000  DensityUnits=kg/m^3  Mass=smiData.Solid(11).mass  MassUnits=kg  CenterOfMass=smiData.Solid(11).CoM  CenterOfMassUnits=mm  MomentsOfInertia=smiData.Solid(11).MoI  MomentsOfInertiaUnits=kg*mm^2  ProductsOfInertia=smiData.Solid(11).PoI  ProductsOfInertiaUnits=kg*mm^2  GraphicType=FromGeometry  MarkerShape=Sphere  MarkerSize=10  GraphicVisPropType=SimpleVisualProperties  GraphicDiffuseColor=smiData.Solid(11).color  GraphicOpacity=smiData.Solid(11).opacity  GraphicSpecularColor=[0.5 0.5 0.5 1.0]  GraphicAmbientColor=[0.15 0.15 0.15 1.0]  GraphicEmissiveColor=[0.0 0.0 0.0 1.0]  GraphicShininess=75  DoExposeReferenceFrame=on  SerializedFrames=<Frames/>
  F : PMIOPort  Side=Left
  connections:
  Solid/RConn1 -- ReferenceFrame/RConn1 -- F/RConn1

== system Hexapod_PD/Base/Base_Side_a_3_RIGID/MotorStator_2_RIGID ==
  ReferenceFrame : sm_lib/Frames and Transforms/Reference Frame
  Solid : sm_lib/Body Elements/File Solid  ExtGeomFileName=MotorStator_Default_sldprt.STEP  UnitType=FromFile  ExtGeomFileUnits=m  StepReaderType=HEX  ExportConvexHullGeometry=off  InertiaType=Custom  BasedOnType=DensityFromFile  Density=1000  DensityUnits=kg/m^3  Mass=smiData.Solid(11).mass  MassUnits=kg  CenterOfMass=smiData.Solid(11).CoM  CenterOfMassUnits=mm  MomentsOfInertia=smiData.Solid(11).MoI  MomentsOfInertiaUnits=kg*mm^2  ProductsOfInertia=smiData.Solid(11).PoI  ProductsOfInertiaUnits=kg*mm^2  GraphicType=FromGeometry  MarkerShape=Sphere  MarkerSize=10  GraphicVisPropType=SimpleVisualProperties  GraphicDiffuseColor=smiData.Solid(11).color  GraphicOpacity=smiData.Solid(11).opacity  GraphicSpecularColor=[0.5 0.5 0.5 1.0]  GraphicAmbientColor=[0.15 0.15 0.15 1.0]  GraphicEmissiveColor=[0.0 0.0 0.0 1.0]  GraphicShininess=75  DoExposeReferenceFrame=on  SerializedFrames=<Frames/>
  F : PMIOPort  Side=Left
  connections:
  Solid/RConn1 -- ReferenceFrame/RConn1 -- F/RConn1

== system Hexapod_PD/Base/Base_Side_a_3_RIGID/base_plate_corner_connector_mm_1_RIGID ==
  ReferenceFrame : sm_lib/Frames and Transforms/Reference Frame
  Solid : sm_lib/Body Elements/File Solid  ExtGeomFileName=base_plate_corner_connector_mm_Default_sldprt.STEP  UnitType=FromFile  ExtGeomFileUnits=m  StepReaderType=HEX  ExportConvexHullGeometry=off  InertiaType=Custom  BasedOnType=DensityFromFile  Density=1000  DensityUnits=kg/m^3  Mass=smiData.Solid(1).mass  MassUnits=kg  CenterOfMass=smiData.Solid(1).CoM  CenterOfMassUnits=in  MomentsOfInertia=smiData.Solid(1).MoI  MomentsOfInertiaUnits=kg*in^2  ProductsOfInertia=smiData.Solid(1).PoI  ProductsOfInertiaUnits=kg*in^2  GraphicType=FromGeometry  MarkerShape=Sphere  MarkerSize=10  GraphicVisPropType=SimpleVisualProperties  GraphicDiffuseColor=smiData.Solid(1).color  GraphicOpacity=smiData.Solid(1).opacity  GraphicSpecularColor=[0.5 0.5 0.5 1.0]  GraphicAmbientColor=[0.15 0.15 0.15 1.0]  GraphicEmissiveColor=[0.0 0.0 0.0 1.0]  GraphicShininess=75  DoExposeReferenceFrame=on  SerializedFrames=<Frames/>
  F : PMIOPort  Side=Left
  connections:
  Solid/RConn1 -- ReferenceFrame/RConn1 -- F/RConn1

== system Hexapod_PD/Base/Base_Side_a_3_RIGID/base_plate_corner_connector_mm_2_RIGID ==
  ReferenceFrame : sm_lib/Frames and Transforms/Reference Frame
  Solid : sm_lib/Body Elements/File Solid  ExtGeomFileName=base_plate_corner_connector_mm_Default_sldprt.STEP  UnitType=FromFile  ExtGeomFileUnits=m  StepReaderType=HEX  ExportConvexHullGeometry=off  InertiaType=Custom  BasedOnType=DensityFromFile  Density=1000  DensityUnits=kg/m^3  Mass=smiData.Solid(1).mass  MassUnits=kg  CenterOfMass=smiData.Solid(1).CoM  CenterOfMassUnits=in  MomentsOfInertia=smiData.Solid(1).MoI  MomentsOfInertiaUnits=kg*in^2  ProductsOfInertia=smiData.Solid(1).PoI  ProductsOfInertiaUnits=kg*in^2  GraphicType=FromGeometry  MarkerShape=Sphere  MarkerSize=10  GraphicVisPropType=SimpleVisualProperties  GraphicDiffuseColor=smiData.Solid(1).color  GraphicOpacity=smiData.Solid(1).opacity  GraphicSpecularColor=[0.5 0.5 0.5 1.0]  GraphicAmbientColor=[0.15 0.15 0.15 1.0]  GraphicEmissiveColor=[0.0 0.0 0.0 1.0]  GraphicShininess=75  DoExposeReferenceFrame=on  SerializedFrames=<Frames/>
  F : PMIOPort  Side=Left
  connections:
  Solid/RConn1 -- ReferenceFrame/RConn1 -- F/RConn1

== system Hexapod_PD/Base/Base_Side_a_3_RIGID/base_plate_mm_1_RIGID ==
  ReferenceFrame : sm_lib/Frames and Transforms/Reference Frame
  Solid : sm_lib/Body Elements/File Solid  ExtGeomFileName=base_plate_mm_Default_sldprt.STEP  UnitType=FromFile  ExtGeomFileUnits=m  StepReaderType=HEX  ExportConvexHullGeometry=off  InertiaType=Custom  BasedOnType=DensityFromFile  Density=1000  DensityUnits=kg/m^3  Mass=smiData.Solid(8).mass  MassUnits=kg  CenterOfMass=smiData.Solid(8).CoM  CenterOfMassUnits=mm  MomentsOfInertia=smiData.Solid(8).MoI  MomentsOfInertiaUnits=kg*mm^2  ProductsOfInertia=smiData.Solid(8).PoI  ProductsOfInertiaUnits=kg*mm^2  GraphicType=FromGeometry  MarkerShape=Sphere  MarkerSize=10  GraphicVisPropType=SimpleVisualProperties  GraphicDiffuseColor=smiData.Solid(8).color  GraphicOpacity=smiData.Solid(8).opacity  GraphicSpecularColor=[0.5 0.5 0.5 1.0]  GraphicAmbientColor=[0.15 0.15 0.15 1.0]  GraphicEmissiveColor=[0.0 0.0 0.0 1.0]  GraphicShininess=75  DoExposeReferenceFrame=on  SerializedFrames=<Frames/>
  F : PMIOPort  Side=Left
  connections:
  Solid/RConn1 -- ReferenceFrame/RConn1 -- F/RConn1

== system Hexapod_PD/Base/Base_Side_a_3_RIGID/bumper_1_RIGID ==
  ReferenceFrame : sm_lib/Frames and Transforms/Reference Frame
  Solid : sm_lib/Body Elements/File Solid  ExtGeomFileName=bumper_Default_sldprt.STEP  UnitType=FromFile  ExtGeomFileUnits=m  StepReaderType=HEX  ExportConvexHullGeometry=off  InertiaType=Custom  BasedOnType=DensityFromFile  Density=1000  DensityUnits=kg/m^3  Mass=smiData.Solid(7).mass  MassUnits=kg  CenterOfMass=smiData.Solid(7).CoM  CenterOfMassUnits=mm  MomentsOfInertia=smiData.Solid(7).MoI  MomentsOfInertiaUnits=kg*mm^2  ProductsOfInertia=smiData.Solid(7).PoI  ProductsOfInertiaUnits=kg*mm^2  GraphicType=FromGeometry  MarkerShape=Sphere  MarkerSize=10  GraphicVisPropType=SimpleVisualProperties  GraphicDiffuseColor=smiData.Solid(7).color  GraphicOpacity=smiData.Solid(7).opacity  GraphicSpecularColor=[0.5 0.5 0.5 1.0]  GraphicAmbientColor=[0.15 0.15 0.15 1.0]  GraphicEmissiveColor=[0.0 0.0 0.0 1.0]  GraphicShininess=75  DoExposeReferenceFrame=on  SerializedFrames=<Frames/>
  F : PMIOPort  Side=Left
  connections:
  Solid/RConn1 -- ReferenceFrame/RConn1 -- F/RConn1

== system Hexapod_PD/Base/Base_Side_a_3_RIGID/prox_sensor_1_RIGID ==
  ReferenceFrame : sm_lib/Frames and Transforms/Reference Frame
  Solid : sm_lib/Body Elements/File Solid  ExtGeomFileName=prox_sensor_95245A233_sldprt.STEP  UnitType=FromFile  ExtGeomFileUnits=m  StepReaderType=HEX  ExportConvexHullGeometry=off  InertiaType=Custom  BasedOnType=DensityFromFile  Density=1000  DensityUnits=kg/m^3  Mass=smiData.Solid(9).mass  MassUnits=kg  CenterOfMass=smiData.Solid(9).CoM  CenterOfMassUnits=mm  MomentsOfInertia=smiData.Solid(9).MoI  MomentsOfInertiaUnits=kg*mm^2  ProductsOfInertia=smiData.Solid(9).PoI  ProductsOfInertiaUnits=kg*mm^2  GraphicType=FromGeometry  MarkerShape=Sphere  MarkerSize=10  GraphicVisPropType=SimpleVisualProperties  GraphicDiffuseColor=smiData.Solid(9).color  GraphicOpacity=smiData.Solid(9).opacity  GraphicSpecularColor=[0.5 0.5 0.5 1.0]  GraphicAmbientColor=[0.15 0.15 0.15 1.0]  GraphicEmissiveColor=[0.0 0.0 0.0 1.0]  GraphicShininess=75  DoExposeReferenceFrame=on  SerializedFrames=<Frames/>
  F : PMIOPort  Side=Left
  connections:
  Solid/RConn1 -- ReferenceFrame/RConn1 -- F/RConn1

== system Hexapod_PD/Base/Base_Side_a_3_RIGID/prox_sensor_2_RIGID ==
  ReferenceFrame : sm_lib/Frames and Transforms/Reference Frame
  Solid : sm_lib/Body Elements/File Solid  ExtGeomFileName=prox_sensor_95245A233_sldprt.STEP  UnitType=FromFile  ExtGeomFileUnits=m  StepReaderType=HEX  ExportConvexHullGeometry=off  InertiaType=Custom  BasedOnType=DensityFromFile  Density=1000  DensityUnits=kg/m^3  Mass=smiData.Solid(9).mass  MassUnits=kg  CenterOfMass=smiData.Solid(9).CoM  CenterOfMassUnits=mm  MomentsOfInertia=smiData.Solid(9).MoI  MomentsOfInertiaUnits=kg*mm^2  ProductsOfInertia=smiData.Solid(9).PoI  ProductsOfInertiaUnits=kg*mm^2  GraphicType=FromGeometry  MarkerShape=Sphere  MarkerSize=10  GraphicVisPropType=SimpleVisualProperties  GraphicDiffuseColor=smiData.Solid(9).color  GraphicOpacity=smiData.Solid(9).opacity  GraphicSpecularColor=[0.5 0.5 0.5 1.0]  GraphicAmbientColor=[0.15 0.15 0.15 1.0]  GraphicEmissiveColor=[0.0 0.0 0.0 1.0]  GraphicShininess=75  DoExposeReferenceFrame=on  SerializedFrames=<Frames/>
  F : PMIOPort  Side=Left
  connections:
  Solid/RConn1 -- ReferenceFrame/RConn1 -- F/RConn1

== system Hexapod_PD/Base/Base_Side_a_3_RIGID/spacer_1_RIGID ==
  ReferenceFrame : sm_lib/Frames and Transforms/Reference Frame
  Solid : sm_lib/Body Elements/File Solid  ExtGeomFileName=spacer_Default_sldprt.STEP  UnitType=FromFile  ExtGeomFileUnits=m  StepReaderType=HEX  ExportConvexHullGeometry=off  InertiaType=Custom  BasedOnType=DensityFromFile  Density=1000  DensityUnits=kg/m^3  Mass=smiData.Solid(3).mass  MassUnits=kg  CenterOfMass=smiData.Solid(3).CoM  CenterOfMassUnits=mm  MomentsOfInertia=smiData.Solid(3).MoI  MomentsOfInertiaUnits=kg*mm^2  ProductsOfInertia=smiData.Solid(3).PoI  ProductsOfInertiaUnits=kg*mm^2  GraphicType=FromGeometry  MarkerShape=Sphere  MarkerSize=10  GraphicVisPropType=SimpleVisualProperties  GraphicDiffuseColor=smiData.Solid(3).color  GraphicOpacity=smiData.Solid(3).opacity  GraphicSpecularColor=[0.5 0.5 0.5 1.0]  GraphicAmbientColor=[0.15 0.15 0.15 1.0]  GraphicEmissiveColor=[0.0 0.0 0.0 1.0]  GraphicShininess=75  DoExposeReferenceFrame=on  SerializedFrames=<Frames/>
  F : PMIOPort  Side=Left
  connections:
  Solid/RConn1 -- ReferenceFrame/RConn1 -- F/RConn1

== system Hexapod_PD/Base/Base_Side_a_3_RIGID/spacer_2_RIGID ==
  ReferenceFrame : sm_lib/Frames and Transforms/Reference Frame
  Solid : sm_lib/Body Elements/File Solid  ExtGeomFileName=spacer_Default_sldprt.STEP  UnitType=FromFile  ExtGeomFileUnits=m  StepReaderType=HEX  ExportConvexHullGeometry=off  InertiaType=Custom  BasedOnType=DensityFromFile  Density=1000  DensityUnits=kg/m^3  Mass=smiData.Solid(3).mass  MassUnits=kg  CenterOfMass=smiData.Solid(3).CoM  CenterOfMassUnits=mm  MomentsOfInertia=smiData.Solid(3).MoI  MomentsOfInertiaUnits=kg*mm^2  ProductsOfInertia=smiData.Solid(3).PoI  ProductsOfInertiaUnits=kg*mm^2  GraphicType=FromGeometry  MarkerShape=Sphere  MarkerSize=10  GraphicVisPropType=SimpleVisualProperties  GraphicDiffuseColor=smiData.Solid(3).color  GraphicOpacity=smiData.Solid(3).opacity  GraphicSpecularColor=[0.5 0.5 0.5 1.0]  GraphicAmbientColor=[0.15 0.15 0.15 1.0]  GraphicEmissiveColor=[0.0 0.0 0.0 1.0]  GraphicShininess=75  DoExposeReferenceFrame=on  SerializedFrames=<Frames/>
  F : PMIOPort  Side=Left
  connections:
  Solid/RConn1 -- ReferenceFrame/RConn1 -- F/RConn1

== system Hexapod_PD/Base/Base_Side_a_3_RIGID/x1942K49_303_Stainless_Steel_Rigid_Leveling_Mount_with_Nylon_Cushion_1_RIGID ==
  ReferenceFrame : sm_lib/Frames and Transforms/Reference Frame
  Solid : sm_lib/Body Elements/File Solid  ExtGeomFileName=1942K49_303 Stainless Steel Rigid Leveling Mount with Nylon Cushion_1942K49_sldprt.STEP  UnitType=FromFile  ExtGeomFileUnits=m  StepReaderType=HEX  ExportConvexHullGeometry=off  InertiaType=Custom  BasedOnType=DensityFromFile  Density=1000  DensityUnits=kg/m^3  Mass=smiData.Solid(2).mass  MassUnits=kg  CenterOfMass=smiData.Solid(2).CoM  CenterOfMassUnits=in  MomentsOfInertia=smiData.Solid(2).MoI  MomentsOfInertiaUnits=kg*in^2  ProductsOfInertia=smiData.Solid(2).PoI  ProductsOfInertiaUnits=kg*in^2  GraphicType=FromGeometry  MarkerShape=Sphere  MarkerSize=10  GraphicVisPropType=SimpleVisualProperties  GraphicDiffuseColor=smiData.Solid(2).color  GraphicOpacity=smiData.Solid(2).opacity  GraphicSpecularColor=[0.5 0.5 0.5 1.0]  GraphicAmbientColor=[0.15 0.15 0.15 1.0]  GraphicEmissiveColor=[0.0 0.0 0.0 1.0]  GraphicShininess=75  DoExposeReferenceFrame=on  SerializedFrames=<Frames/>
  F : PMIOPort  Side=Left
  connections:
  Solid/RConn1 -- ReferenceFrame/RConn1 -- F/RConn1

== system Hexapod_PD/Base/Base_Side_a_3_RIGID/x90576A137_Medium_Strength_Steel_Nylon_Insert_Locknut_1_RIGID ==
  ReferenceFrame : sm_lib/Frames and Transforms/Reference Frame
  Solid : sm_lib/Body Elements/File Solid  ExtGeomFileName=90576A137_Medium-Strength Steel Nylon-Insert Locknut_90576A137_sldprt.STEP  UnitType=FromFile  ExtGeomFileUnits=m  StepReaderType=HEX  ExportConvexHullGeometry=off  InertiaType=Custom  BasedOnType=DensityFromFile  Density=1000  DensityUnits=kg/m^3  Mass=smiData.Solid(5).mass  MassUnits=kg  CenterOfMass=smiData.Solid(5).CoM  CenterOfMassUnits=mm  MomentsOfInertia=smiData.Solid(5).MoI  MomentsOfInertiaUnits=kg*mm^2  ProductsOfInertia=smiData.Solid(5).PoI  ProductsOfInertiaUnits=kg*mm^2  GraphicType=FromGeometry  MarkerShape=Sphere  MarkerSize=10  GraphicVisPropType=SimpleVisualProperties  GraphicDiffuseColor=smiData.Solid(5).color  GraphicOpacity=smiData.Solid(5).opacity  GraphicSpecularColor=[0.5 0.5 0.5 1.0]  GraphicAmbientColor=[0.15 0.15 0.15 1.0]  GraphicEmissiveColor=[0.0 0.0 0.0 1.0]  GraphicShininess=75  DoExposeReferenceFrame=on  SerializedFrames=<Frames/>
  F : PMIOPort  Side=Left
  connections:
  Solid/RConn1 -- ReferenceFrame/RConn1 -- F/RConn1

== system Hexapod_PD/Base/Base_Side_a_3_RIGID/x90576A137_Medium_Strength_Steel_Nylon_Insert_Locknut_2_RIGID ==
  ReferenceFrame : sm_lib/Frames and Transforms/Reference Frame
  Solid : sm_lib/Body Elements/File Solid  ExtGeomFileName=90576A137_Medium-Strength Steel Nylon-Insert Locknut_90576A137_sldprt.STEP  UnitType=FromFile  ExtGeomFileUnits=m  StepReaderType=HEX  ExportConvexHullGeometry=off  InertiaType=Custom  BasedOnType=DensityFromFile  Density=1000  DensityUnits=kg/m^3  Mass=smiData.Solid(5).mass  MassUnits=kg  CenterOfMass=smiData.Solid(5).CoM  CenterOfMassUnits=mm  MomentsOfInertia=smiData.Solid(5).MoI  MomentsOfInertiaUnits=kg*mm^2  ProductsOfInertia=smiData.Solid(5).PoI  ProductsOfInertiaUnits=kg*mm^2  GraphicType=FromGeometry  MarkerShape=Sphere  MarkerSize=10  GraphicVisPropType=SimpleVisualProperties  GraphicDiffuseColor=smiData.Solid(5).color  GraphicOpacity=smiData.Solid(5).opacity  GraphicSpecularColor=[0.5 0.5 0.5 1.0]  GraphicAmbientColor=[0.15 0.15 0.15 1.0]  GraphicEmissiveColor=[0.0 0.0 0.0 1.0]  GraphicShininess=75  DoExposeReferenceFrame=on  SerializedFrames=<Frames/>
  F : PMIOPort  Side=Left
  connections:
  Solid/RConn1 -- ReferenceFrame/RConn1 -- F/RConn1

== system Hexapod_PD/Base/Base_Side_a_3_RIGID/x90576A137_Medium_Strength_Steel_Nylon_Insert_Locknut_3_RIGID ==
  ReferenceFrame : sm_lib/Frames and Transforms/Reference Frame
  Solid : sm_lib/Body Elements/File Solid  ExtGeomFileName=90576A137_Medium-Strength Steel Nylon-Insert Locknut_90576A137_sldprt.STEP  UnitType=FromFile  ExtGeomFileUnits=m  StepReaderType=HEX  ExportConvexHullGeometry=off  InertiaType=Custom  BasedOnType=DensityFromFile  Density=1000  DensityUnits=kg/m^3  Mass=smiData.Solid(5).mass  MassUnits=kg  CenterOfMass=smiData.Solid(5).CoM  CenterOfMassUnits=mm  MomentsOfInertia=smiData.Solid(5).MoI  MomentsOfInertiaUnits=kg*mm^2  ProductsOfInertia=smiData.Solid(5).PoI  ProductsOfInertiaUnits=kg*mm^2  GraphicType=FromGeometry  MarkerShape=Sphere  MarkerSize=10  GraphicVisPropType=SimpleVisualProperties  GraphicDiffuseColor=smiData.Solid(5).color  GraphicOpacity=smiData.Solid(5).opacity  GraphicSpecularColor=[0.5 0.5 0.5 1.0]  GraphicAmbientColor=[0.15 0.15 0.15 1.0]  GraphicEmissiveColor=[0.0 0.0 0.0 1.0]  GraphicShininess=75  DoExposeReferenceFrame=on  SerializedFrames=<Frames/>
  F : PMIOPort  Side=Left
  connections:
  Solid/RConn1 -- ReferenceFrame/RConn1 -- F/RConn1
